simulink model "quarter_car_passive"  (R2024a)
settings: Solver=ode4  StartTime=0.0  StopTime=8  FixedStep=0.001  RelTol=1e-3
model workspace (MAT data in the model file):
  p.ms = 300
  p.mu = 40
  p.ks = 18000
  p.kt = 180000
  p.cs = 1500
  p.g = 9.81
  p.dt = 0.002
  p.T = 8
  p.travelLimit = 0.06
  qc_road_input = [0 0.002 0.004 0.006 0.008 0.01 0.012 0.014 0.016 0.018 0.02 0.022 ... (8002 elements, 4001x2)]
values from neighbouring files (symbols this model uses):
  p = qc_parameters()    [START_HERE.m]    (also in build_simulink.m; run_studies.m; verify_project.m = qc_parameters(); [A,B]=qc_matrices(p); verify_simulink.m)
settings Model: Creator=k34ga  LastModifiedBy=k34ga

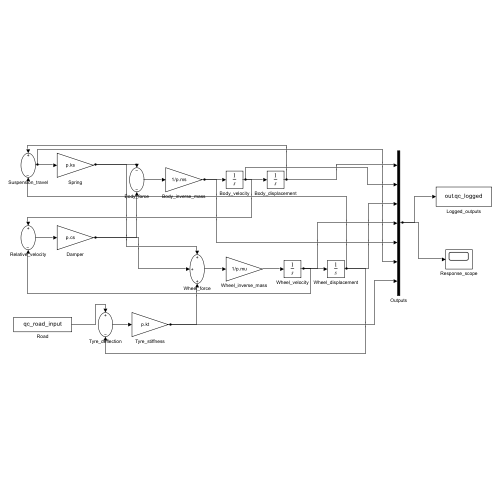
[thumbnail: Simulink's stored preview of the top-level diagram]
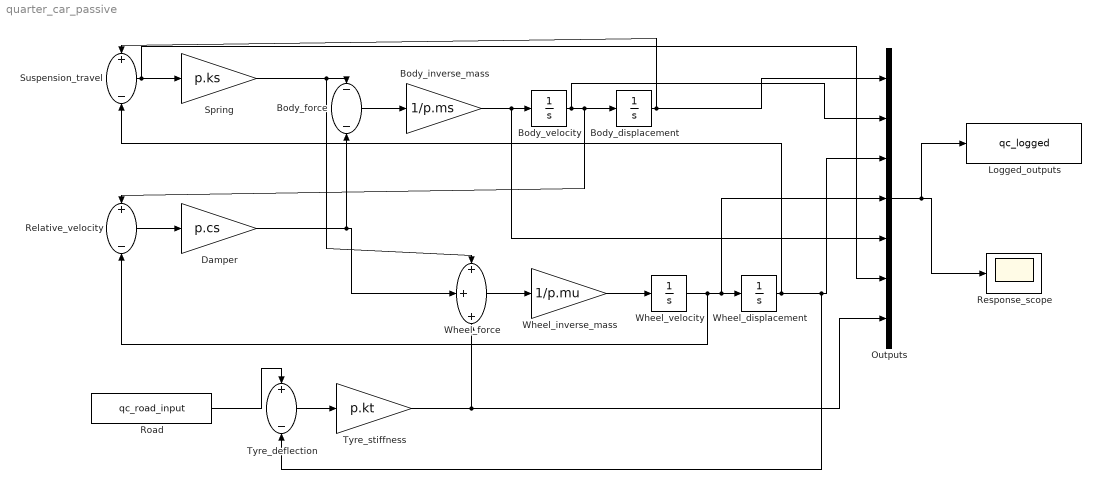
== system quarter_car_passive ==
  Body_displacement : Integrator
  Body_force : Sum  Inputs=--
  Body_inverse_mass : Gain  Gain=1/p.ms
  Body_velocity : Integrator
  Damper : Gain  Gain=p.cs
  Logged_outputs : ToWorkspace  VariableName=qc_logged  SaveFormat=Timeseries  SampleTime=-1
  Outputs : Mux  Inputs=7
  Relative_velocity : Sum  Inputs=+-
  Response_scope : Scope
  Road : FromWorkspace  VariableName=qc_road_input
  Spring : Gain  Gain=p.ks
  Suspension_travel : Sum  Inputs=+-
  Tyre_deflection : Sum  Inputs=+-
  Tyre_stiffness : Gain  Gain=p.kt
  Wheel_displacement : Integrator
  Wheel_force : Sum  Inputs=+++
  Wheel_inverse_mass : Gain  Gain=1/p.mu
  Wheel_velocity : Integrator
  wires:
  Road/1 -> Tyre_deflection/1
  Wheel_displacement/1 -> Tyre_deflection/2, Outputs/3, Suspension_travel/2
  Tyre_deflection/1 -> Tyre_stiffness/1
  Body_displacement/1 -> Suspension_travel/1, Outputs/1
  Suspension_travel/1 -> Spring/1, Outputs/6
  Body_velocity/1 -> Relative_velocity/1, Body_displacement/1, Outputs/2
  Wheel_velocity/1 -> Wheel_displacement/1, Outputs/4, Relative_velocity/2
  Relative_velocity/1 -> Damper/1
  Spring/1 -> Body_force/1, Wheel_force/1
  Damper/1 -> Body_force/2, Wheel_force/2
  Body_force/1 -> Body_inverse_mass/1
  Body_inverse_mass/1 -> Body_velocity/1, Outputs/5
  Tyre_stiffness/1 -> Wheel_force/3, Outputs/7
  Wheel_force/1 -> Wheel_inverse_mass/1
  Wheel_inverse_mass/1 -> Wheel_velocity/1
  Outputs/1 -> Logged_outputs/1, Response_scope/1
